simulink model "FSEA_Vehicle"  (R2026a)
settings: Solver=ode23tb  StopTime=5  FixedStep=.001  RelTol=1e-1
model workspace (MAT data in the model file):
  A_mu = 10
  B_reff = 8.386
  CONVERTER_DATA = [0 0.1 0.2 0.3 0.4 0.5 0.6 0.7 0.8 0.81 0.82 0.83 ... (63 elements, 21x3)]
  Cps = 2
  Cz = 7766.25
  DOWN_TABLE = [0 0 0 0 0 0 5 5 7.5 7.5 15 15 ... (30 elements, 6x5)]
  DOWN_TH_BP = [0 5 40 50 90 100]
  D_reff = 0.25826
  EMAP = [-40 215 245 264 264 267 267 267 267 267 -44 117 ... (110 elements, 10x11)]
  F0z = [6086.4 4324.8]
  F_reff = 0.07394
  F_zmax = 10000
  F_zmin = 100
  F_zo = 4000
  Kz = 48000
  MF : object (value not decoded)
  NCyl = 6
  NE_VEC = [800 1200 1600 2000 2400 2800 3200 3600 4000 4400 4800]
  Pstd = 101325
  Rair = 287
  SUS : object (value not decoded)
  TH_VEC = [0; 20; 30; 40; 50; 60; 70; 80; 90; 100]
  TWAITdn = 1.25
  TWAITup = 0.1
  Tin = [1 2 3 4 5 6 7 8 9 10 2 2 ... (20 elements, 10x2)]
  Tstd = 293.15
  UP_TABLE = [7.5 7.5 15 25 40 40 25 25 35 45 70 80 ... (30 elements, 6x5)]
  UP_TH_BP = [0 25 35 50 90 100]
  VEH : object (value not decoded)
  V_o = 16.7
  V_xlow = 1
  Vd = 0.00346
  WH : object (value not decoded)
  a = 1.515
  alpha_max = 1.5
  alpha_min = -1.5
  b = 1.504
  c_zo = 209651
  epsilon = 0.1
  f_air = [0 0 0 0 0 0 0 0 0 0 0 0 ... (256 elements, 16x16)]
  f_co = [0 0 0 0 0 0 0 0 0 0 0 0 ... (256 elements, 16x16)]
  f_co2 = [0 0 0 0 0 0 0 0 0 0 0 0 ... (256 elements, 16x16)]
  f_eff = [352.135682859 352.135682859 320.724378192 303.655312657 295.930136708 291.240087194 291.240271258 291.240312459 291.240275452 291.240198499 291.240100781 291.240018769 ... (256 elements, 16x16)]
  f_fuel = [0 0 0 0 0 0 0 0 0 0 0 0 ... (256 elements, 16x16)]
  f_hc = [0 0 0 0 0 0 0 0 0 0 0 0 ... (256 elements, 16x16)]
  f_nox = [0 0 0 0 0 0 0 0 0 0 0 0 ... (256 elements, 16x16)]
  f_pm = [0 0 0 0 0 0 0 0 0 0 0 0 ... (256 elements, 16x16)]
  f_susp_axl_bp = [1 2]
  f_susp_dz_bp = [-4 -0.14 -0.13 -0.12 -0.11 -0.1 -0.09 -0.08 -0.07 -0.06 -0.05 -0.04 ... (31 elements, 1x31)]
  f_susp_dzdot_bp = [-4 -0.14 -0.13 -0.12 -0.11 -0.1 -0.09 -0.08 -0.07 -0.06 -0.05 -0.04 ... (31 elements, 1x31)]
  f_susp_fmz = [-213379.591456 -28099.591456 -27619.591456 -27139.591456 -26659.591456 -26179.591456 -25699.591456 -25219.591456 -24739.591456 -24259.591456 -23779.591456 -23299.591456 ... (468968 elements, 31x31x61x2x4)]
  f_susp_geom = [-0.832564012244 0.043269987756 0.045538987756 0.047807987756 0.050076987756 0.052345987756 0.054614987756 0.056883987756 0.059152987756 0.061421987756 0.063690987756 0.065959987756 ... (11346 elements, 31x61x2x3)]
  f_susp_strgdelta_bp = [-0.523598775598 -0.506145483078 -0.488692190558 -0.471238898038 -0.453785605519 -0.436332312999 -0.418879020479 -0.401425727959 -0.383972435439 -0.366519142919 -0.349065850399 -0.331612557879 ... (61 elements, 1x61)]
  f_tbrake = [0 76.8593923996 105.140482948 131.533638111 157.926793274 176.658631717 176.65727296 176.656856686 176.656879077 176.657093756 176.657404516 176.65772406 ... (256 elements, 16x16)]
  f_tbrake_n_bpt = [0 649.519052838 912.419621844 1175.32019085 1438.22075986 1701.12132886 1964.02189787 2226.92246687 2489.82303588 2752.72360489 3015.62417389 3278.5247429 ... (16 elements, 1x16)]
  f_tbrake_t_bpt = [0 34.6410161514 61.0341713143 87.4273264773 113.82048164 140.213636803 166.606791966 192.999947129 219.393102292 245.786257455 272.179412618 298.572567781 ... (16 elements, 1x16)]
  f_texh = [766.752464599 766.752464599 786.17542386 801.679939032 884.591982581 910.574397722 910.571871054 910.570774534 910.570601632 910.570821151 910.571247242 910.571639815 ... (256 elements, 16x16)]
  f_twc_eff_co = [0.17 0.25 0.45 0.99 0.99 0.99 0.99]
  f_twc_eff_hc = [0.21 0.375 0.75 0.98 0.98 0.98 0.98]
  f_twc_eff_lam = [0.909090909 0.944055944 0.979020979 1 1.013986014 1.048951049 1.083916084]
  f_twc_eff_nox = [0.98 0.98 0.98 0.97 0.05 0.02 0]
  h = 0.134
  k_z = 50
  kappa_max = 1.5
  kappa_min = -1.5
  lam_Cx = 1
  lam_Cy = 1
  lam_Cz = 1
  lam_Ex = 1
  lam_Ey = 1
  lam_F_zo = 1
  lam_Hx = 1
  lam_Hy = 1
  lam_Kxkappa = 1
  lam_Kyalpha = 1
  lam_Kygamma = 1
  lam_Kzgamma = 1
  lam_Mr = 1
  lam_Mx = 1
  lam_My = 1
  lam_S = 1
  lam_VMx = 1
  lam_Vx = 1
  lam_Vy = 1
  lam_Vykappa = 1
  lam_muV = 0
  lam_mux = 1
  lam_muy = 1
  lam_t = 1
  lam_xalpha = 1
  lam_ykappa = 1
  numWheel = 4
  p_Cx1 = 1.579
  p_Cy1 = 1.3332
  p_Dx1 = 1.0422
  p_Dx2 = -0.08285
  p_Dx3 = 0
  p_Dy1 = 0.8784
  p_Dy2 = -0.06445
  p_Dy3 = 0
  p_Ex1 = 0.11185
  p_Ex2 = 0.3127
  p_Ex3 = 0
  p_Ex4 = 0.001603
  p_Ey1 = -0.8227
  p_Ey2 = -0.6062
  p_Ey3 = 0.09825
  p_Ey4 = -6.546
  p_Ey5 = 0
  p_Fz1 = 0.7098
  p_Hx1 = 0.00021585
  p_Hx2 = 0.0011538
  p_Hy1 = -0.0018043
  p_Hy2 = 0.003518
  p_Kx1 = 21.69
  p_Kx2 = 13.774
  p_Kx3 = -0.4119
  p_Ky1 = -15.314
  p_Ky2 = 1.7044
  p_Ky3 = 0.36986
  p_Ky4 = 1.9896
  p_Ky5 = 0
  p_Ky6 = -0.9004
  p_Ky7 = -0.2328
  p_Vx1 = 1.5973e-05
  p_Vx2 = 0.0001043
  p_Vy1 = -0.006642
  p_Vy2 = 0.03597
  p_Vy3 = -0.1621
  p_Vy4 = -0.4908
  p_pmx1 = 0
  p_px1 = -0.3489
  p_px2 = 0.382
  p_px3 = -0.09634
  p_px4 = 0.06447
  p_py1 = -0.6249
  p_py2 = -0.06535
  p_py3 = -0.1668
  p_py4 = 0.2834
  p_py5 = 0
  path : object (value not decoded)
  pio = 220000
  q_Fcx = 0
  q_Fz2 = 15.4
  q_Fzy = 0
  q_reo = 0.9974
  q_sx1 = -0.007764
  q_sx10 = 0.2824
  q_sx11 = 5.349
  q_sx12 = 0
  q_sx13 = 0
  q_sx14 = 0
  q_sx2 = 1.1915
  q_sx3 = 0.013948
  q_sx4 = 4.912
  q_sx5 = 1.02
  q_sx6 = 22.83
  q_sx7 = 0.7104
  q_sx8 = -0.023393
  q_sx9 = 0.6581
  q_sy1 = 0.00702
  q_sy2 = 0
  q_sy3 = 0.001515
  q_sy4 = 8.514e-05
  q_sy5 = 0
  q_sy6 = 0
  q_sy7 = 0.9008
  q_sy8 = -0.4089
  q_v1 = 0.0007742
  q_v2 = 0.04667
  r_Bx1 = 12.531
  r_Bx2 = 9.532
  r_Bx3 = 0
  r_By1 = 10.615
  r_By2 = 7.705
  r_By3 = 3.433e-06
  r_By4 = 0
  r_Cx1 = 1.019
  r_Cy1 = 1.0585
  r_Ex1 = -0.4487
  r_Ex2 = -0.4726
  r_Ey1 = 0.3132
  r_Ey2 = 7.63e-06
  r_Hx1 = 0.0002374
  r_Hy1 = 0.011646
  r_Hy2 = 7.63e-06
  r_Vy1 = 0.05654
  r_Vy2 = 7.63e-06
  r_Vy3 = 0
  r_Vy4 = 99.9
  r_Vy5 = 2
  r_Vy6 = 15.814
  r_o = 0.3135
  reqTmaxT = [nan 0.285774810084 0.647179872268 nan nan nan nan nan nan nan nan nan ... (168 elements, 21x8)]
  vehSpd = [0 2.77777777778 5.55555555556 8.33333333333 11.1111111111 13.8888888889 16.6666666667 19.4444444444 22.2222222222 25 27.7777777778 30.5555555556 ... (21 elements, 1x21)]
  vehWidth = 2
  w = 1
symbols that are objects in the model workspace (value not decoded): VEH
undefined symbols (not defined in the file or in its folder): InertFrm
libraries: sharedtransform x6, vehdynlibtirecommon x2, vehdynlibtire x2, autolibutils x2, autolibshared x2
(part 4 of 4)

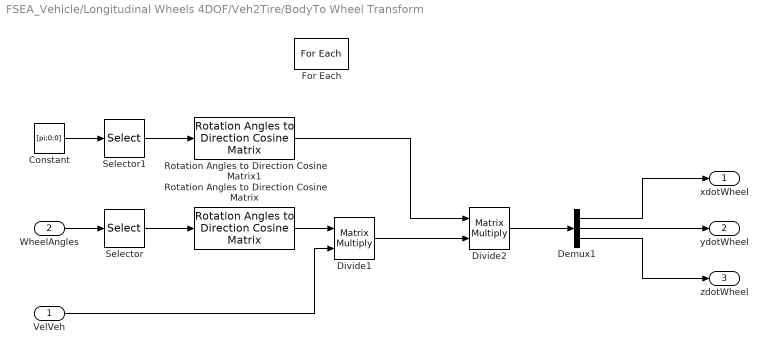
== system FSEA_Vehicle/Longitudinal Wheels 4DOF/Veh2Tire/BodyTo Wheel Transform ==
  VelVeh : Inport  Partition=on  PartitionDimension=2  PartitionWidth=1  PartitionOffset=0
  WheelAngles : Inport  Port=2  Partition=on  PartitionDimension=2  PartitionWidth=1  PartitionOffset=0
  Constant : Constant  Value=[pi;0;0]
  Demux1 : Demux  Outputs=3
  Divide1 : Product  Inputs=**  Multiplication=Matrix(*)
  Divide2 : Product  Inputs=**  Multiplication=Matrix(*)
  For Each : ForEach  DisableCoverage=on
  Rotation Angles to Direction Cosine Matrix : sharedtransform/Rotation Angles to Direction Cosine Matrix  rotationOrder=ZYX  aMode=2
  Rotation Angles to Direction Cosine Matrix1 : sharedtransform/Rotation Angles to Direction Cosine Matrix  rotationOrder=ZYX  aMode=2
  Selector : Selector  InputPortWidth=3  IndexOptions=Index vector (dialog)  Indices=[3 2 1]  OutputSizes=1
  Selector1 : Selector  InputPortWidth=3  IndexOptions=Index vector (dialog)  Indices=[3 2 1]  OutputSizes=1
  xdotWheel : Outport  ConcatenationDimension=1  VectorParamsAs1DForOutWhenUnconnected=off
  ydotWheel : Outport  Port=2  ConcatenationDimension=1  VectorParamsAs1DForOutWhenUnconnected=off
  zdotWheel : Outport  Port=3  ConcatenationDimension=1  VectorParamsAs1DForOutWhenUnconnected=off
  wires:
  Divide2/1 -> Demux1/1
  Demux1/1 -> xdotWheel/1
  Demux1/2 -> ydotWheel/1
  Demux1/3 -> zdotWheel/1
  Rotation Angles to Direction Cosine Matrix/1 -> Divide1/1
  VelVeh/1 -> Divide1/2
  WheelAngles/1 -> Selector/1
  Selector/1 -> Rotation Angles to Direction Cosine Matrix/1
  Selector1/1 -> Rotation Angles to Direction Cosine Matrix1/1
  Rotation Angles to Direction Cosine Matrix1/1 -> Divide2/1
  Divide1/1 -> Divide2/2
  Constant/1 -> Selector1/1

== system FSEA_Vehicle/Longitudinal Wheels 4DOF/Velocity and Vertical Load/Bicycle ==
  VehFdbk : Inport
  Bicycle Fz : Subsystem
  Bicycle V : Subsystem
  VehVel : Outport  PortDimensions=[3,4]  VectorParamsAs1DForOutWhenUnconnected=off
  Fz : Outport  Port=2  VectorParamsAs1DForOutWhenUnconnected=off
  wires:
  VehFdbk/1 -> Bicycle V/1(In1), Bicycle Fz/1(VehFdbk)
  Bicycle V/1(Out1) -> VehVel/1
  Bicycle Fz/1(Out1) -> Fz/1

== system FSEA_Vehicle/Longitudinal Wheels 4DOF/Velocity and Vertical Load/Dual ==
  VehFdbk : Inport
  Dual Fz : Subsystem
  Dual V : Subsystem
  VehVel : Outport  VectorParamsAs1DForOutWhenUnconnected=off
  Fz : Outport  Port=2  VectorParamsAs1DForOutWhenUnconnected=off
  wires:
  Dual V/1(Out1) -> VehVel/1
  VehFdbk/1 -> Dual Fz/1(In1), Dual V/1(In1)
  Dual Fz/1(Out1) -> Fz/1

== system FSEA_Vehicle/Longitudinal Wheels 4DOF/Axle Forces/Bicycle/Wheel Angles ==
  Front : Inport
  Camber : Inport  Port=2
  Constant : Constant  Value=zeros(4,1)
  Reshape : Reshape  OutputDimensionality=Row vector (2-D)
  Reshape1 : Reshape  OutputDimensionality=Row vector (2-D)
  Reshape2 : Reshape  OutputDimensionality=Row vector (2-D)
  Vector Concatenate3 : Concatenate  NumInputs=3  Mode=Multidimensional array
  Vehicle : Outport  VectorParamsAs1DForOutWhenUnconnected=off
  wires:
  Reshape/1 -> Vector Concatenate3/3
  Reshape2/1 -> Vector Concatenate3/2
  Vector Concatenate3/1 -> Vehicle/1
  Reshape1/1 -> Vector Concatenate3/1
  Front/1 -> Reshape/1
  Camber/1 -> Reshape1/1
  Constant/1 -> Reshape2/1

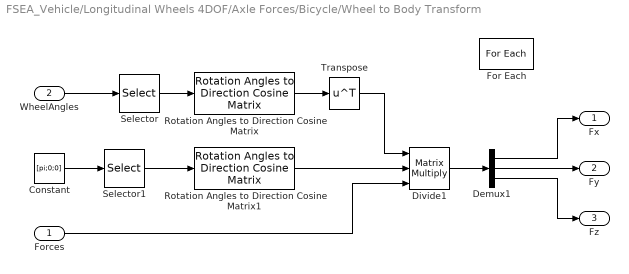
== system FSEA_Vehicle/Longitudinal Wheels 4DOF/Axle Forces/Bicycle/Wheel to Body Transform ==
  Forces : Inport  PortDimensions=[3,1]  Partition=on  PartitionDimension=2  PartitionWidth=1  PartitionOffset=0
  WheelAngles : Inport  Port=2  Partition=on  PartitionDimension=2  PartitionWidth=1  PartitionOffset=0
  Constant : Constant  Value=[pi;0;0]
  Demux1 : Demux  Outputs=3
  Divide1 : Product  Inputs=***  Multiplication=Matrix(*)
  For Each : ForEach  DisableCoverage=on
  Rotation Angles to Direction Cosine Matrix : sharedtransform/Rotation Angles to Direction Cosine Matrix  rotationOrder=ZYX  aMode=2
  Rotation Angles to Direction Cosine Matrix1 : sharedtransform/Rotation Angles to Direction Cosine Matrix  rotationOrder=ZYX  aMode=2
  Selector : Selector  InputPortWidth=3  IndexOptions=Index vector (dialog)  Indices=[3 2 1]  OutputSizes=1
  Selector1 : Selector  InputPortWidth=3  IndexOptions=Index vector (dialog)  Indices=[3 2 1]  OutputSizes=1
  Transpose : Math  Operator=transpose
  Fx : Outport  ConcatenationDimension=1  VectorParamsAs1DForOutWhenUnconnected=off
  Fy : Outport  Port=2  ConcatenationDimension=1  VectorParamsAs1DForOutWhenUnconnected=off
  Fz : Outport  Port=3  ConcatenationDimension=1  VectorParamsAs1DForOutWhenUnconnected=off
  wires:
  Demux1/1 -> Fx/1
  Demux1/2 -> Fy/1
  Demux1/3 -> Fz/1
  Forces/1 -> Divide1/3
  WheelAngles/1 -> Selector/1
  Selector/1 -> Rotation Angles to Direction Cosine Matrix/1
  Rotation Angles to Direction Cosine Matrix1/1 -> Divide1/2
  Divide1/1 -> Demux1/1
  Selector1/1 -> Rotation Angles to Direction Cosine Matrix1/1
  Constant/1 -> Selector1/1
  Rotation Angles to Direction Cosine Matrix/1 -> Transpose/1
  Transpose/1 -> Divide1/1

== system FSEA_Vehicle/Longitudinal Wheels 4DOF/Axle Forces/Dual/Wheel Angles ==
  Front : Inport
  Camber : Inport  Port=2
  Constant : Constant  Value=zeros(4,1)
  Reshape : Reshape  OutputDimensionality=Row vector (2-D)
  Reshape1 : Reshape  OutputDimensionality=Row vector (2-D)
  Reshape2 : Reshape  OutputDimensionality=Row vector (2-D)
  Vector Concatenate3 : Concatenate  NumInputs=3  Mode=Multidimensional array
  Vehicle : Outport  VectorParamsAs1DForOutWhenUnconnected=off
  wires:
  Reshape/1 -> Vector Concatenate3/3
  Reshape2/1 -> Vector Concatenate3/2
  Vector Concatenate3/1 -> Vehicle/1
  Reshape1/1 -> Vector Concatenate3/1
  Constant/1 -> Reshape2/1
  Camber/1 -> Reshape1/1
  Front/1 -> Reshape/1

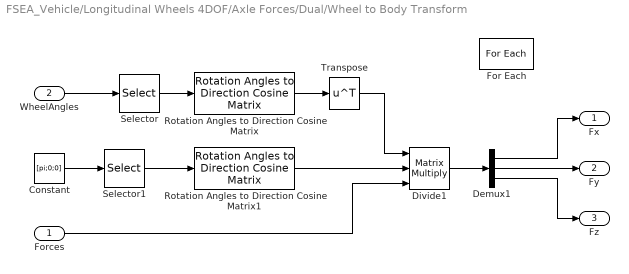
== system FSEA_Vehicle/Longitudinal Wheels 4DOF/Axle Forces/Dual/Wheel to Body Transform ==
  Forces : Inport  PortDimensions=[3,1]  Partition=on  PartitionDimension=2  PartitionWidth=1  PartitionOffset=0
  WheelAngles : Inport  Port=2  Partition=on  PartitionDimension=2  PartitionWidth=1  PartitionOffset=0
  Constant : Constant  Value=[pi;0;0]
  Demux1 : Demux  Outputs=3
  Divide1 : Product  Inputs=***  Multiplication=Matrix(*)
  For Each : ForEach  DisableCoverage=on
  Rotation Angles to Direction Cosine Matrix : sharedtransform/Rotation Angles to Direction Cosine Matrix  rotationOrder=ZYX  aMode=2
  Rotation Angles to Direction Cosine Matrix1 : sharedtransform/Rotation Angles to Direction Cosine Matrix  rotationOrder=ZYX  aMode=2
  Selector : Selector  InputPortWidth=3  IndexOptions=Index vector (dialog)  Indices=[3 2 1]  OutputSizes=1
  Selector1 : Selector  InputPortWidth=3  IndexOptions=Index vector (dialog)  Indices=[3 2 1]  OutputSizes=1
  Transpose : Math  Operator=transpose
  Fx : Outport  ConcatenationDimension=1  VectorParamsAs1DForOutWhenUnconnected=off
  Fy : Outport  Port=2  ConcatenationDimension=1  VectorParamsAs1DForOutWhenUnconnected=off
  Fz : Outport  Port=3  ConcatenationDimension=1  VectorParamsAs1DForOutWhenUnconnected=off
  wires:
  Demux1/1 -> Fx/1
  Demux1/2 -> Fy/1
  Demux1/3 -> Fz/1
  Forces/1 -> Divide1/3
  WheelAngles/1 -> Selector/1
  Selector/1 -> Rotation Angles to Direction Cosine Matrix/1
  Rotation Angles to Direction Cosine Matrix1/1 -> Divide1/2
  Divide1/1 -> Demux1/1
  Selector1/1 -> Rotation Angles to Direction Cosine Matrix1/1
  Constant/1 -> Selector1/1
  Rotation Angles to Direction Cosine Matrix/1 -> Transpose/1
  Transpose/1 -> Divide1/1

== system FSEA_Vehicle/Longitudinal Wheels 4DOF/Tires/MF/scale factors with friction ==
  lamda_mu_x : Inport
  lamda_mu_y : Inport  Port=2
  0 : Constant  Value=[zeros(1,numWheels)]  VectorParams1D=off
  Reshape : Reshape  OutputDimensionality=Row vector (2-D)  OutputDimensions=[1,numWheels]
  Reshape1 : Reshape  OutputDimensionality=Row vector (2-D)  OutputDimensions=[1,numWheels]
  Signal Specification3 : SignalSpecification  Unit=1
  Vector Concatenate : Concatenate  NumInputs=5  Mode=Multidimensional array
  ones : Constant  Value=[ones(23,numWheels)]  VectorParams1D=off
  ones2 : Constant  Value=ones(1,numWheels)  VectorParams1D=off
  lambdas : Outport  Unit=1  VectorParamsAs1DForOutWhenUnconnected=off
  wires:
  lamda_mu_y/1 -> Reshape1/1
  lamda_mu_x/1 -> Reshape/1
  ones2/1 -> Vector Concatenate/1  "lambda_Fz0"
  Vector Concatenate/1 -> Signal Specification3/1
  ones/1 -> Vector Concatenate/5
  0/1 -> Vector Concatenate/4  "lamda_mu_V"
  Reshape1/1 -> Vector Concatenate/3
  Reshape/1 -> Vector Concatenate/2
  Signal Specification3/1 -> lambdas/1

== system FSEA_Vehicle/Longitudinal Wheels 4DOF/Velocity and Vertical Load/Bicycle/Bicycle Fz ==
  Bus Element In1 : Inport  PortName=VehFdbk
  Add : Sum
  Bus Selector : BusSelector  OutputSignals=BdyFrm.Forces.Tires.FrntTire.Fz,BdyFrm.Forces.Tires.RearTire.Fz
  Cont LPF : autolibutils/Cont LPF  wc=100*2*pi*ones(4,1)  AbsoluteTolerance=auto  aMode=2
  Saturation : Saturate  UpperLimit=10e3*ones(4,1)  LowerLimit=100*ones(4,1)  ZeroCross=off
  Unsprung Mass : Constant  Value=[0 0 80 80].*9.81
  Vector Concatenate : Concatenate  NumInputs=4
  Out1 : Outport  PortDimensions=4  VectorParamsAs1DForOutWhenUnconnected=off
  wires:
  Vector Concatenate/1 -> Saturation/1
  Saturation/1 -> Cont LPF/1
  Cont LPF/1 -> Add/1
  Bus Element In1/1 -> Bus Selector/1
  Bus Selector/1 -> Vector Concatenate/2, Vector Concatenate/1  "<Fz>"
  Bus Selector/2 -> Vector Concatenate/3, Vector Concatenate/4  "<Fz>"
  Unsprung Mass/1 -> Add/2
  Add/1 -> Out1/1

== system FSEA_Vehicle/Longitudinal Wheels 4DOF/Velocity and Vertical Load/Bicycle/Bicycle V ==
  In1 : Inport
  Bus Selector : BusSelector  OutputSignals=BdyFrm.FrntAxl.Vel.xdot,BdyFrm.FrntAxl.Vel.ydot,BdyFrm.FrntAxl.Vel.zdot
  Bus Selector3 : BusSelector  OutputSignals=BdyFrm.RearAxl.Vel.xdot,BdyFrm.RearAxl.Vel.ydot,BdyFrm.RearAxl.Vel.zdot
  Mux : Mux  Inputs=3
  Mux1 : Mux  Inputs=3
  Vector Concatenate1 : Concatenate  NumInputs=4  Mode=Multidimensional array  ConcatenateDimension=2
  Out1 : Outport  PortDimensions=[3,4]  VectorParamsAs1DForOutWhenUnconnected=off
  wires:
  Bus Selector3/1 -> Mux1/1  "<xdot>"
  Mux/1 -> Vector Concatenate1/2, Vector Concatenate1/1
  In1/1 -> Bus Selector3/1, Bus Selector/1
  Bus Selector/1 -> Mux/1  "<xdot>"
  Mux1/1 -> Vector Concatenate1/4, Vector Concatenate1/3
  Vector Concatenate1/1 -> Out1/1
  Bus Selector/2 -> Mux/2  "<ydot>"
  Bus Selector/3 -> Mux/3  "<zdot>"
  Bus Selector3/2 -> Mux1/2  "<ydot>"
  Bus Selector3/3 -> Mux1/3  "<zdot>"

== system FSEA_Vehicle/Longitudinal Wheels 4DOF/Velocity and Vertical Load/Dual/Dual Fz ==
  In1 : Inport
  Add : Sum
  Bus Selector6 : BusSelector  OutputSignals=BdyFrm.Forces.Tires.FrntTires.Lft.Fz,BdyFrm.Forces.Tires.FrntTires.Rght.Fz,BdyFrm.Forces.Tires.RearTires.Lft.Fz,BdyFrm.Forces.Tires.RearTires.Rght.Fz
  Cont LPF : autolibutils/Cont LPF  wc=100*2*pi  AbsoluteTolerance=auto  aMode=2
  Saturation : Saturate  UpperLimit=10e3  LowerLimit=100  ZeroCross=off
  Unsprung Mass : Constant  Value=[0 0 0 0]
  Vector Concatenate : Concatenate  NumInputs=4
  Out1 : Outport  VectorParamsAs1DForOutWhenUnconnected=off
  wires:
  In1/1 -> Bus Selector6/1
  Saturation/1 -> Cont LPF/1
  Cont LPF/1 -> Add/1
  Vector Concatenate/1 -> Saturation/1
  Bus Selector6/2 -> Vector Concatenate/2  "<Fz>"
  Bus Selector6/1 -> Vector Concatenate/1  "<Fz>"
  Bus Selector6/3 -> Vector Concatenate/3  "<Fz>"
  Bus Selector6/4 -> Vector Concatenate/4  "<Fz>"
  Add/1 -> Out1/1
  Unsprung Mass/1 -> Add/2

== system FSEA_Vehicle/Longitudinal Wheels 4DOF/Velocity and Vertical Load/Dual/Dual V ==
  In1 : Inport
  Bus Selector1 : BusSelector  OutputSignals=BdyFrm.FrntAxl.Lft.Vel.xdot,BdyFrm.FrntAxl.Lft.Vel.ydot,BdyFrm.FrntAxl.Lft.Vel.zdot  OutputAsBus=on
  Bus Selector2 : BusSelector  OutputSignals=BdyFrm.FrntAxl.Rght.Vel.xdot,BdyFrm.FrntAxl.Rght.Vel.ydot,BdyFrm.FrntAxl.Rght.Vel.zdot  OutputAsBus=on
  Bus Selector4 : BusSelector  OutputSignals=BdyFrm.RearAxl.Lft.Vel.xdot,BdyFrm.RearAxl.Lft.Vel.ydot,BdyFrm.RearAxl.Lft.Vel.zdot  OutputAsBus=on
  Bus Selector5 : BusSelector  OutputSignals=BdyFrm.RearAxl.Rght.Vel.xdot,BdyFrm.RearAxl.Rght.Vel.ydot,BdyFrm.RearAxl.Rght.Vel.zdot  OutputAsBus=on
  Bus to Vector{5..8} (4 alike) : BusToVector
  Vector Concatenate2 : Concatenate  NumInputs=4  Mode=Multidimensional array  ConcatenateDimension=2
  Out1 : Outport  VectorParamsAs1DForOutWhenUnconnected=off
  wires:
  Bus to Vector6/1 -> Vector Concatenate2/2
  Bus Selector2/1 -> Bus to Vector6/1
  Bus to Vector8/1 -> Vector Concatenate2/4
  Bus Selector4/1 -> Bus to Vector7/1
  Bus to Vector5/1 -> Vector Concatenate2/1
  Bus Selector1/1 -> Bus to Vector5/1
  In1/1 -> Bus Selector1/1, Bus Selector2/1, Bus Selector4/1, Bus Selector5/1
  Bus Selector5/1 -> Bus to Vector8/1
  Bus to Vector7/1 -> Vector Concatenate2/3
  Vector Concatenate2/1 -> Out1/1

== matlab function FSEA_Vehicle/Vehicle Signal Routing/Single Track Vehicle Signal Routing/For 3D Visualization ==
  data: angles output size=3; angleIn input size=3; GeomXYZ output size=3; GemoXYZIn input size=3; Ground input size=4; trackW parameter; wheelB parameter
function [angles,GeomXYZ]= three26(angleIn, GemoXYZIn, Ground,trackW, wheelB)%#codegen
coder.allowpcode('plain')
% Copyright 2018 The MathWorks, Inc.
[angles,GeomXYZ]= vdynthree2six(angleIn, GemoXYZIn, Ground,trackW, wheelB);

== matlab function FSEA_Vehicle/Vehicle Signal Routing/Dual Track Vehicle Signal Routing/For 3D Visualization ==
  data: angles output size=3; angleIn input size=3; GeomXYZ output size=3; GemoXYZIn input size=3; Ground input size=4; trackW parameter; wheelB parameter
function [angles,GeomXYZ]= three26(angleIn, GemoXYZIn, Ground,trackW, wheelB)%#codegen
coder.allowpcode('plain')
% Copyright 2018 The MathWorks, Inc.
[angles,GeomXYZ]= vdynthree2six(angleIn, GemoXYZIn, Ground,trackW, wheelB);
